simulink model "Dll_Control_AFO_V8_5_R2019b"  (R2019b)
settings: Solver=ode2  StartTime=0.0  StopTime=10  FixedStep=Ts  RelTol=1e-3
InitFcn:
  | modelDir=fileparts(get_param(bdroot,'FileName'));addpath(modelDir);rootDir=fileparts(modelDir);if isfolder(rootDir),addpath(rootDir);end;fmuDir=fullfile(rootDir,'fmu');if isfolder(fmuDir),addpath(fmuDir);end;if evalin('base','exist(''Wf0'',''var'')'),assignin('base','Wfb',evalin('base','Wf0'));end;
values from neighbouring files (symbols this model uses):
  A80 = 0.10573    [RunCtrlSysModelSHT.m]
  b11 = B(1,1)*1    [RunCtrlSysModelSHT.m]
  b21 = B(2,1)*1    [RunCtrlSysModelSHT.m]
  d31 = D(3,1)    [RunCtrlSysModelSHT.m]
  d41 = D(4,1)    [RunCtrlSysModelSHT.m]
  ExternalSecondaryAirEnabled = 0    [RunCtrlSysModelSHT.m]
  InitAir = zeros(50,1)    [RunCtrlSysModelSHT.m]
  Mkg0 = 0    [RunCtrlSysModelSHT.m]
  MkpDirectCommand = Mkp0    (= 999.278795578)    [RunCtrlSysModelSHT.m]
  MkpMax = 1200    [RunCtrlSysModelSHT.m]
  Ng0 = 38000    [RunCtrlSysModelSHT.m]
  NgMax = Ng0*1.05    (= 39900)    [RunCtrlSysModelSHT.m]
  Np0 = 20800    [RunCtrlSysModelSHT.m]
  NpDem = Np0    (= 20800)    [RunCtrlSysModelSHT.m]
  omega_u = 20    [RunCtrlSysModelSHT.m]
  power0 = 2176600    [RunCtrlSysModelSHT.m]
  RotorLoadCfg = struct(      'designNpRpm', Np0,      'designPowerW', power0,      'thetaZeroDeg', 0,      'thetaDesignDeg', 12,      'profileTorqueFraction', 0.15,      'thetaValidRangeDeg', [6, 14])    [RunCtrlSysModelSHT.m]
  RotorLoadInputMode = 'legacyPower'    [RunCtrlSysModelSHT.m]
  T45Max = 1400    [RunCtrlSysModelSHT.m]
  ThetaCommandDeg = RotorLoadCfg.thetaDesignDeg    [RunCtrlSysModelSHT.m]
  Ts = 0.025    [RunCtrlSysModelSHT.m]
  Wf0 = 0.151914044493225    (= 0.151914044493)    [RunCtrlSysModelSHT.m]
  WfMax = Wf0*2    (= 0.303828088986)    [RunCtrlSysModelSHT.m]
  WfMin = Wf0*0.01    (= 0.00151914044493)    [RunCtrlSysModelSHT.m]
  WfRateLim = 1.5    [RunCtrlSysModelSHT.m]
undefined symbols (not defined in the file or in its folder): sigbuilder_block, Wfb
libraries: simulink x10
(part 1 of 4)
settings Model: Creator=Jiangjc21  LastModifiedBy=k_liu
settings SolverCC: NumberNewtonIterations=10  SolverJacobianMethodControl=FullPerturbation
settings DataIOCC: ReturnWorkspaceOutputs=off

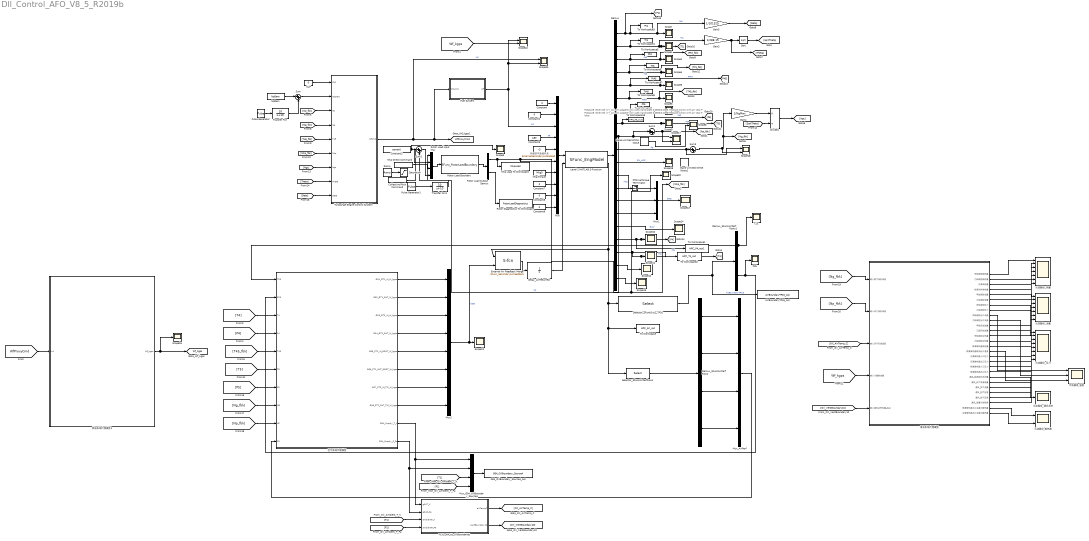
== system Dll_Control_AFO_V8_5_R2019b ==
  note: PsealA/B reserved (V7_22). Oil adapter still uses hardcoded 3.08e5/3.20e5. Replace Const with air seal P later.
  note: PsealA/B reserved (V7_22). Oil adapter still uses hardcoded 3.08e5/3.20e5. Replace Const with air seal P later.
  AirBoundaryTP16_out : ToWorkspace  VariableName=AirBoundaryTP16_out  SampleTime=-1
  Band-Limited White Noise : simulink/Sources/Band-Limited White Noise  Cov=[0.1]  Ts=Ts  seed=[23341]
  Band-Limited White Noise1 : simulink/Sources/Band-Limited White Noise  Cov=[0.1]  Ts=Ts  seed=[23341]
  CLP : Constant  Value=0
  Collective Pitch Command : Constant  Value=ThetaCommandDeg
  Constant{,1,7..9} (5 alike) : Constant  Value=0
  Constant2 : Constant  Value=power0
  Constant3 : Constant  Value=A80
  Delay_AirReturn50 : UnitDelay  InitialCondition=InitAir  SampleTime=Ts  HasFrameUpgradeWarning=on
  Demux : Demux  Outputs=20
  Demux_SFuncAirPerfRows : Demux
  Demux_SFuncAirPerfRows1 : Demux  Outputs=2
  Divide1 : Product  Inputs=*/
  External Air Feedback Merge : M-S-Function  FunctionName=SFunc_SecondaryAirFeedback
  FCN_G04_to_OilBoundaries : MATLAB Function  TreatAsAtomicUnit=on
  Fuel System : Subsystem
  G04_OilBoundary_Source4_out : ToWorkspace  VariableName=G04_OilBoundary_Source4  SampleTime=-1
  Gain3 : Gain  Gain=1/288.15
  Gain4 : Gain  Gain=1/NgMax
  Gain5 : Gain  Gain=1/101325
  Level-2 MATLAB S-Function : M-S-Function  FunctionName=SFunc_EngModel  Parameters=InitStat, InitOut, InitAir
  Mkg Torque : Constant  Value=Mkg0
  Mkp Direct Command : Constant  Value=MkpDirectCommand
  Mkp Load To Workspace : ToWorkspace  VariableName=MkpLoad  SaveFormat=Structure With Time  SampleTime=-1
  Mux : Mux  Inputs=10
  Mux1 : Mux  Inputs=3
  Mux2 : Mux  Inputs=8
  Mux_AirPerf : Mux
  Mux_G04_OilBoundary_Source4 : Mux
  NpDem : Constant  Value=NpDem
  P25 : Scope
  PTDriveTorque Terminator : Terminator
  Pulse Generator : DiscretePulseGenerator  PulseType=Time based  Amplitude=-2000  Period=100  PulseWidth=5  PhaseDelay=1
  Pulse Generator1 : DiscretePulseGenerator  PulseType=Time based  Amplitude=-4  Period=10  PulseWidth=50  PhaseDelay=1
  Ramp : simulink/Sources/Ramp  slope=-1e6  start=0  InitialOutput=0
  Rotor Diagnostics To Workspace : ToWorkspace  VariableName=RotorLoadDiagnostics  SaveFormat=Structure With Time  SampleTime=-1
  Rotor Load Boundary : M-S-Function  FunctionName=SFunc_RotorLoadBoundary  Parameters=RotorLoadInputMode,RotorLoadCfg
  Rotor Load Input Mux : Mux
  Rotor Load Output Demux : Demux  Outputs=[1 5]
  Saturation : Saturate  UpperLimit=0  LowerLimit=-power0*0.9
  Scope{,1..16,19..21} (20 alike) : Scope
  Scope{17..18,22,25} (4 alike) : Scope  NumInputPorts=2
  Selector_SFuncAirPerfRows : Selector  InputPortWidth=50  IndexOptions=Index vector (dialog)  Indices=[23 24 33 34]  OutputSizes=4
  Selector_SFuncOut2_TP16 : Selector  InputPortWidth=50  IndexOptions=Index vector (dialog)  Indices=[33 34 ]  OutputSizes=1
  Sqrt : Sqrt  SaturateOnIntegerOverflow=on
  Sum{,1..3} (4 alike) : Sum  Inputs=|++
  T25 : Scope
  To Workspace : ToWorkspace  VariableName=HPC_air_out  SaveFormat=Timeseries  SampleTime=-1
  To Workspace1 : ToWorkspace  VariableName=HPC_P4_out1  SaveFormat=Timeseries  SampleTime=-1
  To Workspace13 : ToWorkspace  VariableName=HPC_T5_out1  SaveFormat=Timeseries  SampleTime=-1
  To Workspace2 : ToWorkspace  VariableName=HPC_T4_out  SaveFormat=Timeseries  SampleTime=-1
  To Workspace3 : ToWorkspace  VariableName=Pt1  SaveFormat=Timeseries  SampleTime=-1
  To Workspace4 : ToWorkspace  VariableName=Tt1  SaveFormat=Timeseries  SampleTime=-1
  To Workspace5 : ToWorkspace  VariableName=Pt3  SaveFormat=Timeseries  SampleTime=-1
  To Workspace6 : ToWorkspace  VariableName=Tt3  SaveFormat=Timeseries  SampleTime=-1
  To Workspace7 : ToWorkspace  VariableName=Pt45  SaveFormat=Timeseries  SampleTime=-1
  To Workspace8 : ToWorkspace  VariableName=Tt45  SaveFormat=Timeseries  SampleTime=-1
  To Workspace9 : ToWorkspace  VariableName=Pt5  SaveFormat=Timeseries  SampleTime=-1
  Transfer Fcn : TransferFcn  Numerator=[10]  Denominator=[1 10]
  Transfer Fcn1 : TransferFcn  Numerator=[10]  Denominator=[1 10]
  Turboshaft Engine Control System : Subsystem
  外部空气系统开关 : Constant  Value=ExternalSecondaryAirEnabled
  滑油系统代理模型 : Subsystem
  燃油系统代理模型1 : Subsystem
  示波器组_压力 : Scope  NumInputPorts=8
  示波器组_散热器 : Scope  NumInputPorts=2
  示波器组_流量 : Scope  NumInputPorts=7
  示波器组_温度 : Scope  NumInputPorts=3
  示波器组_热量 : Scope  NumInputPorts=7
  示波器组_通风状态 : Scope
  空气系统代理模型 : Subsystem
  tag scope: WfProxyCmd=global, Wf_kgps=global
  wires:
  Demux/5 -> [P45], Scope5/1, To Workspace7/1  "Pt45"
  Mux1/1 -> Scope13/1  "beta"
  [Np_fbk] -> Turboshaft Engine Control System/3(Np)
  外部空气系统开关/1 -> Mux/5
  [Deta] -> Turboshaft Engine Control System/9(Deta)
  [Theta] -> Turboshaft Engine Control System/8(Theta)
  Gain5/1 -> [Deta]
  Demux/7 -> [P5], Scope7/1, To Workspace9/1  "Pt5"
  Divide1/1 -> [Ngc]
  [T45_fbk] -> Turboshaft Engine Control System/5(T45)
  Sqrt/1 -> [SqrtTheta]
  [Ngc] -> Turboshaft Engine Control System/7(Ngc)
  [Ng_fbk] -> Turboshaft Engine Control System/4(Ng)
  [Mkp_fbk] -> Turboshaft Engine Control System/6(Mkp)
  Demux/14 -> Mux1/2
  Demux/2 -> To Workspace4/1, [T1], Scope1/1, Gain3/1  "Tt1"
  Demux/15 -> Mux1/3
  Demux/4 -> [Tt3_fbk], Scope4/1, To Workspace6/1  "Tt3"
  Mux/1 -> Level-2 MATLAB S-Function/1
  Demux/3 -> To Workspace5/1, [Pt3_fbk], Scope2/1  "Pt3"
  Demux/6 -> Scope6/1, [T45_fbk], To Workspace8/1  "Tt45"
  Demux/1 -> [P1], Gain5/1, Scope/1, To Workspace3/1  "Pt1"
  Constant1/1 -> Mux/2
  Demux/8 -> [T5], Scope9/1, To Workspace13/1  "Tt5"
  Demux/11 -> Scope19/1  "SM_HPC"
  Constant9/1 -> Mux/10
  Constant3/1 -> Mux/4  "A8"
  Demux/10 -> Scope18/1, Sum3/1  "Ng"
  Demux/9 -> Sum2/1, Scope17/1, Rotor Load Input Mux/1  "Np"
  Gain4/1 -> Divide1/1
  Constant8/1 -> Mux/9
  Gain3/1 -> [Theta], Sqrt/1
  [SqrtTheta] -> Divide1/2
  Demux/13 -> Mux1/1
  Constant/1 -> Mux/1
  CLP/1 -> Turboshaft Engine Control System/1(CLP)
  Constant7/1 -> Mux/8
  Band-Limited White Noise/1 -> Scope8/1
  Sum2/1 -> Scope17/2, [Np_fbk]
  Sum3/1 -> Scope18/2, Gain4/1, [Ng_fbk]
  Sum/1 -> Turboshaft Engine Control System/2(NpDem)
  Fuel System/1(Wf) -> Mux/3, Scope22/1, Scope25/2  "Wf"
  NpDem/1 -> Sum/1
  Pulse Generator/1 -> Transfer Fcn/1
  Pulse Generator1/1 -> Transfer Fcn1/1
  Ramp/1 -> Saturation/1
  Transfer Fcn/1 -> Sum/2
  Demux/16 -> Scope14/1  "Error"
  Demux/17 -> [P4], Scope10/1, To Workspace1/1  "Pt4"
  Demux/18 -> [T4], Scope11/1, To Workspace2/1  "Tt4"
  Demux/19 -> Scope12/1
  Demux/20 -> Scope15/1
  燃油系统代理模型1/1(Wf_kgps) -> [Wf_kgps], Scope16/1
  Level-2 MATLAB S-Function/1 -> Demux/1
  Level-2 MATLAB S-Function/2 -> Selector_SFuncOut2_TP16/1, To Workspace/1, Selector_SFuncAirPerfRows/1, External Air Feedback Merge/1
  Selector_SFuncOut2_TP16/1 -> AirBoundaryTP16_out/1, Demux_SFuncAirPerfRows1/1  "AirBoundaryTP16"
  Demux_SFuncAirPerfRows1/2 -> 空气系统代理模型/2(P25), P25/1
  [T4] -> 空气系统代理模型/3(T4)
  [P4] -> 空气系统代理模型/4(P4)
  [T45_fbk] -> 空气系统代理模型/5(T45)
  [T5] -> 空气系统代理模型/6(T5)
  [P5] -> 空气系统代理模型/7(P5)
  [Ng_fbk] -> 空气系统代理模型/8(NG)
  [Np_fbk] -> 空气系统代理模型/9(NP)
  空气系统代理模型/1(G01_GT1_IN_W_kgps) -> Mux2/1
  空气系统代理模型/2(G02_GT1_OUT_W_kgps) -> Mux2/2
  空气系统代理模型/3(G03_GT2_IN_W_kgps) -> Mux2/3
  空气系统代理模型/4(G04_GT2_OUT_W_kgps) -> Mux2/4
  空气系统代理模型/5(G05_PT1_IN_ROOT_W_kgps) -> Mux2/5
  空气系统代理模型/6(G06_PT1_OUT_ROOT_W_kgps) -> Mux2/6
  空气系统代理模型/7(G07_PT2_IN_TIP_W_kgps) -> Mux2/7
  空气系统代理模型/8(G08_PT2_OUT_TIP_W_kgps) -> Mux2/8
  Mux2/1 -> Scope21/1, External Air Feedback Merge/2  "beta"
  Selector_SFuncAirPerfRows/1 -> Demux_SFuncAirPerfRows/1
  Demux_SFuncAirPerfRows/2 -> Mux_AirPerf/2
  Delay_AirReturn50/1 -> Level-2 MATLAB S-Function/2
  Demux_SFuncAirPerfRows/1 -> Mux_AirPerf/1
  Demux_SFuncAirPerfRows/3 -> Mux_AirPerf/3
  Demux_SFuncAirPerfRows/4 -> Mux_AirPerf/4
  Mux_AirPerf/1 -> 空气系统代理模型/10(25)
  [Ng_fbk] -> 滑油系统代理模型/1(输入燃气涡轮转速)
  [Np_fbk] -> 滑油系统代理模型/2(输入动力涡轮转速)
  [Wf_kgps] -> 滑油系统代理模型/4(输入计量燃油量)
  [T1] -> FCN_G04_to_OilBoundaries/3(ambientT_K)
  [P1] -> FCN_G04_to_OilBoundaries/4(ambientP_Pa)
  FCN_G04_to_OilBoundaries/1(airTempC) -> [Oil_AirTemp_C]
  FCN_G04_to_OilBoundaries/2(ventBoundary10) -> [Oil_VentBoundary10]
  [T1] -> Mux_G04_OilBoundary_Source4/3
  [P1] -> Mux_G04_OilBoundary_Source4/4
  Mux_G04_OilBoundary_Source4/1 -> G04_OilBoundary_Source4_out/1
  [Oil_AirTemp_C] -> 滑油系统代理模型/3(输入空气系统温度)
  [Oil_VentBoundary10] -> 滑油系统代理模型/5(输入通风边界向量_PaK)
  空气系统代理模型/10(G04_Supply_P_Pa) -> Mux_G04_OilBoundary_Source4/2, FCN_G04_to_OilBoundaries/2(g04P_Pa)
  空气系统代理模型/9(G04_Supply_T_K) -> FCN_G04_to_OilBoundaries/1(g04T_K), Mux_G04_OilBoundary_Source4/1
  滑油系统代理模型/1(甲轴承腔换热量) -> 示波器组_热量/1
  滑油系统代理模型/2(乙轴承腔换热量) -> 示波器组_热量/2
  滑油系统代理模型/3(空滑换热量) -> 示波器组_热量/3
  滑油系统代理模型/4(机匣附件换热量) -> 示波器组_热量/4
  滑油系统代理模型/13(甲轴承腔生热量) -> 示波器组_热量/5
  滑油系统代理模型/14(乙轴承腔生热量) -> 示波器组_热量/6
  滑油系统代理模型/15(燃滑散热器换热量) -> 示波器组_热量/7
  滑油系统代理模型/5(甲轴承腔流量) -> 示波器组_流量/1
  滑油系统代理模型/6(乙轴承腔流量) -> 示波器组_流量/2
  滑油系统代理模型/11(甲腔回油流量) -> 示波器组_流量/3
  滑油系统代理模型/12(乙腔回油流量) -> 示波器组_流量/4
  滑油系统代理模型/22(通风_封严泄漏流量) -> 示波器组_流量/5
  滑油系统代理模型/23(通风_排气流量) -> 示波器组_流量/6
  滑油系统代理模型/26(通风_质量守恒残差) -> 示波器组_流量/7
  滑油系统代理模型/7(甲轴承腔压力) -> 示波器组_压力/1
  滑油系统代理模型/8(乙轴承腔压力) -> 示波器组_压力/2
  滑油系统代理模型/17(空滑散热器入口压力) -> 示波器组_压力/3
  滑油系统代理模型/18(空滑散热器出口压力) -> 示波器组_压力/4
  滑油系统代理模型/19(燃滑散热器入口压力) -> 示波器组_压力/5
  滑油系统代理模型/20(燃滑散热器出口压力) -> 示波器组_压力/6
  滑油系统代理模型/24(通风_封严压差) -> 示波器组_压力/7
  滑油系统代理模型/25(通风_排气压差) -> 示波器组_压力/8
  滑油系统代理模型/9(甲轴承腔出口油温) -> 示波器组_温度/1
  滑油系统代理模型/10(乙轴承腔出口油温) -> 示波器组_温度/2
  滑油系统代理模型/16(燃滑散热器燃油出口温度) -> 示波器组_温度/3
  滑油系统代理模型/21(通风_轴承腔状态向量) -> 示波器组_通风状态/1
  滑油系统代理模型/27(燃滑散热器出口油温与散热量) -> 示波器组_散热器/1
  滑油系统代理模型/28(空滑散热器出口油温与散热量) -> 示波器组_散热器/2
  Constant2/1 -> Rotor Load Input Mux/2, Scope3/1
  Mkp Direct Command/1 -> Rotor Load Input Mux/3
  Collective Pitch Command/1 -> Sum1/1
  Transfer Fcn1/1 -> Sum1/2
  Sum1/1 -> Rotor Load Input Mux/4
  Rotor Load Input Mux/1 -> Rotor Load Boundary/1
  Rotor Load Boundary/1 -> Rotor Load Output Demux/1
  Rotor Load Output Demux/1 -> [Mkp_fbk], Scope20/1, Mux/6, Mkp Load To Workspace/1
  Rotor Load Output Demux/2 -> Rotor Diagnostics To Workspace/1
  Demux/12 -> PTDriveTorque Terminator/1  "Mkp"
  Mkg Torque/1 -> Mux/7
  External Air Feedback Merge/1 -> Delay_AirReturn50/1
  Turboshaft Engine Control System/1(Wfcmd) -> [WfProxyCmd], Fuel System/1(Wf_cmd), Scope25/1  "Wf"
  Demux_SFuncAirPerfRows1/1 -> T25/1, 空气系统代理模型/1(T25)
  [WfProxyCmd] -> 燃油系统代理模型1/1(In1)
  [Wf_kgps] -> Scope22/2

== system Dll_Control_AFO_V8_5_R2019b/Fuel System ==
  Wf_cmd : Inport
  Constant : Constant  Value=Wf0
  Gain3 : Gain  Gain=25
  Integrator3 : Integrator  InitialConditionSource=external  InitialCondition=Wfb  LimitOutput=on  UpperSaturationLimit=WfMax  LowerSaturationLimit=WfMin
  Saturation : Saturate  UpperLimit=WfRateLim  LowerLimit=-WfRateLim
  Sum3 : Sum  Inputs=|+-
  Wf : Outport
  wires:
  Saturation/1 -> Integrator3/1
  Gain3/1 -> Saturation/1
  Sum3/1 -> Gain3/1
  Wf_cmd/1 -> Sum3/1
  Integrator3/1 -> Wf/1, Sum3/2
  Constant/1 -> Integrator3/2

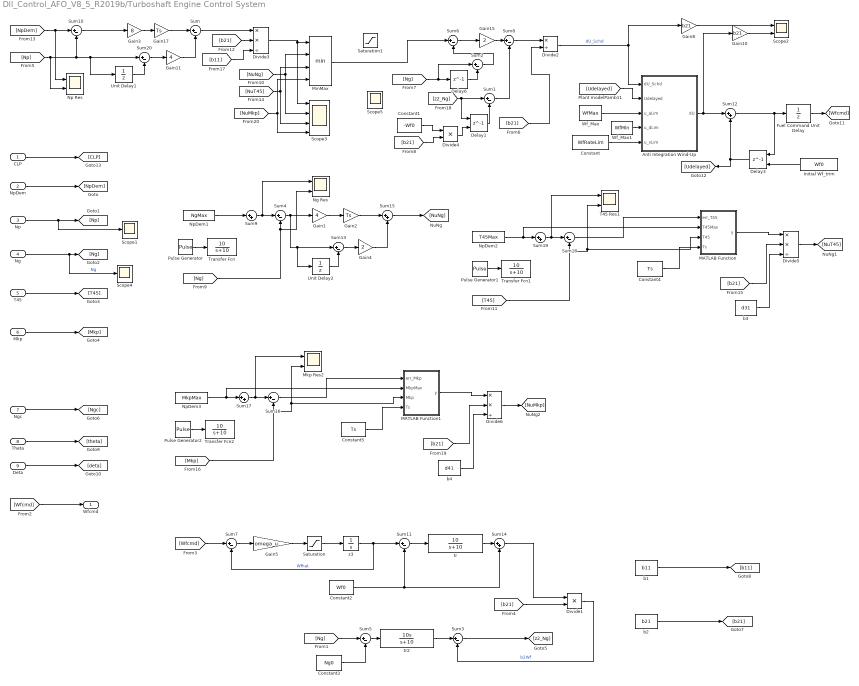
== system Dll_Control_AFO_V8_5_R2019b/Turboshaft Engine Control System ==
  CLP : Inport
  NpDem : Inport  Port=2
  Np : Inport  Port=3
  Ng : Inport  Port=4
  T45 : Inport  Port=5
  Mkp : Inport  Port=6
  Ngc : Inport  Port=7
  Theta : Inport  Port=8
  Deta : Inport  Port=9
  Anti Integration Wind-Up : MATLAB Function  TreatAsAtomicUnit=on
  Constant : Constant  Value=WfRateLim
  Constant1 : Constant  Value=-Wf0
  Constant2 : Constant  Value=Wf0
  Constant3 : Constant  Value=Ng0
  Constant4 : Constant  Value=Ts
  Constant5 : Constant  Value=Ts
  Delay1 : Delay  DelayLength=1  InitialConditionSource=Input port  InitialCondition=Ng0  SampleTime=Ts
      settings: InputPortMap=u0,p4
  Delay3 : Delay  DelayLength=1  InitialConditionSource=Input port  InitialCondition=Wfb  SampleTime=Ts
      settings: InputPortMap=u0,p4
  Delay6 : Delay  DelayLength=1  InitialCondition=Ng0  SampleTime=Ts
  Divide1 : Product  Inputs=**
  Divide2 : Product  Inputs=*/
  Divide3 : Product  Inputs=**/
  Divide4 : Product  Inputs=**
  Divide5 : Product  Inputs=**/
  Divide6 : Product  Inputs=**/
  Fuel Command Unit Delay : UnitDelay  InitialCondition=Wf0  SampleTime=Ts  HasFrameUpgradeWarning=on
  Gain1 : Gain  Gain=4
  Gain10 : Gain  Gain=b21
  Gain11 : Gain  Gain=4
  Gain15 : Gain  Gain=2
  Gain17 : Gain  Gain=Ts
  Gain2 : Gain  Gain=Ts
  Gain3 : Gain  Gain=8
  Gain4 : Gain  Gain=2
  Gain5 : Gain  Gain=omega_u
  Gain8 : Gain  Gain=b21
  Initial Wf_trim : Constant  Value=Wf0
  MATLAB Function : MATLAB Function  TreatAsAtomicUnit=on
  MATLAB Function1 : MATLAB Function  TreatAsAtomicUnit=on
  MinMax : MinMax  Inputs=4
  Mkp Res2 : Scope  NumInputPorts=2
  Ng Res : Scope  NumInputPorts=2
  Np Res : Scope  NumInputPorts=2
  NpDem1 : Constant  Value=NgMax
  NpDem2 : Constant  Value=T45Max
  NpDem3 : Constant  Value=MkpMax
  Pulse Generator : DiscretePulseGenerator  PulseType=Time based  Amplitude=-200  Period=10  PulseWidth=40  PhaseDelay=2
  Pulse Generator1 : DiscretePulseGenerator  PulseType=Time based  Amplitude=-5  Period=10  PulseWidth=40  PhaseDelay=2
  Pulse Generator2 : DiscretePulseGenerator  PulseType=Time based  Amplitude=-50  Period=10  PulseWidth=40  PhaseDelay=2
  Saturation : Saturate  UpperLimit=WfRateLim  LowerLimit=-WfRateLim
  Saturation1 : Saturate  UpperLimit=1000  LowerLimit=-1000
  Scope1 : Scope
  Scope2 : Scope  NumInputPorts=2
  Scope3 : Scope  NumInputPorts=4
  Scope4 : Scope
  Scope5 : Scope  NumInputPorts=2
  Sum{,1..8,10..11,13,16,18,20} (15 alike) : Sum  Inputs=|+-
  Sum{9,12,14..15,17,19} (6 alike) : Sum  Inputs=|++
  T45 Res1 : Scope  NumInputPorts=2
  Transfer Fcn : TransferFcn  Numerator=[10]  Denominator=[1 10]
  Transfer Fcn1 : TransferFcn  Numerator=[10]  Denominator=[1 10]
  Transfer Fcn2 : TransferFcn  Numerator=[10]  Denominator=[1 10]
  Unit Delay1 : UnitDelay  InitialCondition=Np0  SampleTime=-1  HasFrameUpgradeWarning=on
  Unit Delay2 : UnitDelay  InitialCondition=NgMax-Ng0  SampleTime=-1  HasFrameUpgradeWarning=on
  Wf_Max : Constant  Value=WfMax
  Wf_Max1 : Constant  Value=WfMin
  b1 : Constant  Value=b11
  b2 : Constant  Value=b21
  b3 : Constant  Value=d31
  b4 : Constant  Value=d41
  tr : TransferFcn  Numerator=[10]  Denominator=[1 10]
  tr2 : TransferFcn  Numerator=[10 0]  Denominator=[1 10]
  z3 : Integrator  InitialCondition=Wf0
  Wfcmd : Outport
  wires:
  NpDem/1 -> [NpDem]
  Np/1 -> Scope1/1, [Np]
  Ng/1 -> Scope4/1, [Ng]  "Ng"
  T45/1 -> [T45]
  Mkp/1 -> [Mkp]
  [Wfcmd] -> Wfcmd/1
  Ngc/1 -> [Ngc]
  Theta/1 -> [theta]
  Deta/1 -> [deta]
  Delay3/1 -> [Udelayed], Sum12/2
  Initial Wf_trim/1 -> Delay3/2
  Wf_Max1/1 -> Anti Integration Wind-Up/4(u_dLim)
  Wf_Max/1 -> Anti Integration Wind-Up/3(u_aLim)
  CLP/1 -> [CLP]
  z3/1 -> Sum11/1, Sum7/2  "Wfhat"
  Sum7/1 -> Gain5/1
  Constant/1 -> Anti Integration Wind-Up/5(u_vLim)
  [b21] -> Divide2/2
  Anti Integration Wind-Up/1(dU) -> Gain10/1, Sum12/1
  Constant2/1 -> Sum14/2, Sum11/2
  Sum11/1 -> tr/1
  tr/1 -> Sum14/1
  [NpDem] -> Sum10/1, Np Res/1
  Sum8/1 -> Divide2/1
  Gain5/1 -> Saturation/1
  Saturation/1 -> z3/1
  [Wfcmd] -> Sum7/1
  [Udelayed] -> Anti Integration Wind-Up/2(Udelayed)
  Gain8/1 -> Scope2/1
  Gain10/1 -> Scope2/2
  [Np] -> Sum20/1, Unit Delay1/1, Sum10/2, Np Res/2
  tr2/1 -> Sum3/1
  [b21] -> Divide1/2
  Constant3/1 -> Sum5/2
  [Ng] -> Sum5/1
  Sum5/1 -> tr2/1
  Divide1/1 -> Sum3/2  "b2Wf"
  Sum3/1 -> [z2_Ng]
  Sum14/1 -> Divide1/1
  Sum/1 -> Divide3/1
  Gain3/1 -> Gain17/1
  Sum6/1 -> Gain15/1
  Sum20/1 -> Gain11/1
  Unit Delay1/1 -> Sum20/2
  [b21] -> Divide3/2
  [b11] -> Divide3/3
  Divide2/1 -> Anti Integration Wind-Up/1(dU_Schd), Gain8/1  "dU_Schd"
  Gain15/1 -> Sum8/1
  Gain17/1 -> Sum/1
  Gain11/1 -> Sum/2
  [Ng] -> Sum2/1, Delay6/1
  Delay6/1 -> Sum2/2
  b1/1 -> [b11]
  b2/1 -> [b21]
  [z2_Ng] -> Sum1/1, Delay1/1
  Delay1/1 -> Sum1/2
  Constant1/1 -> Divide4/1
  [b21] -> Divide4/2
  Divide4/1 -> Delay1/2
  Sum12/1 -> Fuel Command Unit Delay/1, Delay3/1
  Fuel Command Unit Delay/1 -> [Wfcmd]
  Pulse Generator/1 -> Transfer Fcn/1
  NpDem1/1 -> Sum9/1
  Sum9/1 -> Sum4/1, Ng Res/1
  Gain1/1 -> Gain2/1
  Unit Delay2/1 -> Sum13/2
  Sum13/1 -> Gain4/1
  Sum4/1 -> Unit Delay2/1, Sum13/1, Gain1/1
  Gain2/1 -> Sum15/1
  Divide3/1 -> Scope3/1, MinMax/1
  [NuNg] -> MinMax/2, Scope3/2
  Pulse Generator1/1 -> Transfer Fcn1/1
  NpDem2/1 -> MATLAB Function/2(T45Max), Sum19/1
  Sum19/1 -> Sum18/1, T45 Res1/1
  [T45] -> MATLAB Function/3(T45), T45 Res1/2, Sum18/2
  [b21] -> Divide5/2
  b3/1 -> Divide5/3
  Sum2/1 -> Sum6/2
  Sum1/1 -> Sum8/2
  [NuT45] -> Scope3/3, MinMax/3
  [Ng] -> Ng Res/2, Sum4/2
  Gain4/1 -> Sum15/2
  Sum18/1 -> MATLAB Function/1(err_T45)
  Divide5/1 -> [NuT45]
  MATLAB Function/1(y) -> Divide5/1
  Constant4/1 -> MATLAB Function/4(Ts)
  Sum15/1 -> [NuNg]
  Pulse Generator2/1 -> Transfer Fcn2/1
  Constant5/1 -> MATLAB Function1/4(Ts)
  MATLAB Function1/1(y) -> Divide6/1
  b4/1 -> Divide6/3
  Sum17/1 -> Sum16/1, Mkp Res2/1
  Sum16/1 -> MATLAB Function1/1(err_Mkp)
  NpDem3/1 -> MATLAB Function1/2(MkpMax), Sum17/1
  Divide6/1 -> [NuMkp]
  [b21] -> Divide6/2
  [Mkp] -> MATLAB Function1/3(Mkp), Mkp Res2/2, Sum16/2
  [NuMkp] -> MinMax/4, Scope3/4
  MinMax/1 -> Sum6/1
  Sum10/1 -> Gain3/1

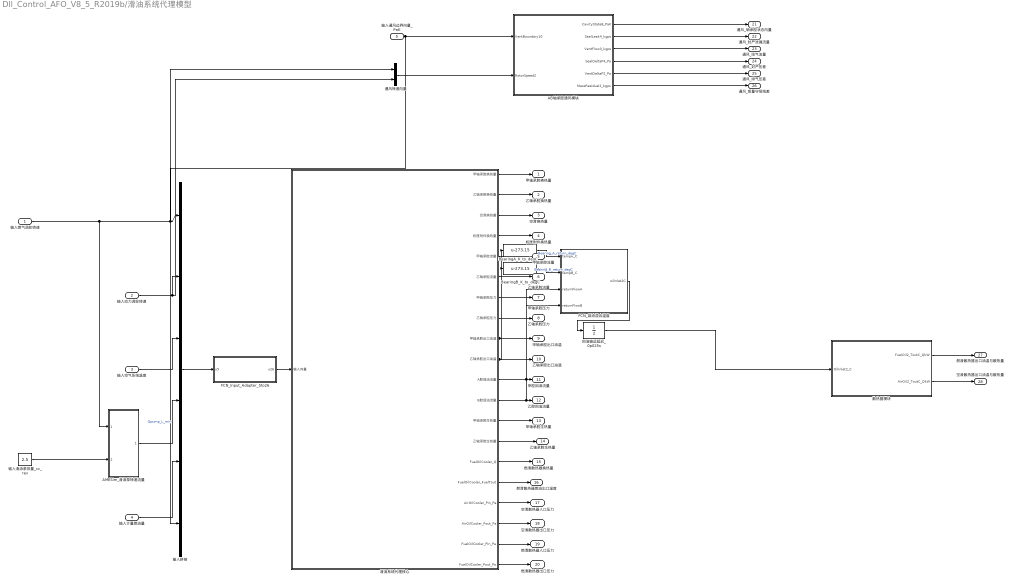
== system Dll_Control_AFO_V8_5_R2019b/滑油系统代理模型 ==
  输入燃气涡轮转速 : Inport
  输入动力涡轮转速 : Inport  Port=2
  输入空气系统温度 : Inport  Port=3
  输入计量燃油量 : Inport  Port=4
  输入通风边界向量_PaK : Inport  Port=5  PortDimensions=10
  AB轴承腔通风模块 : Subsystem
  AMESim_滑油泵转速流量 : Subsystem
  BearingA_K_to_degC : Bias  Description=轴承出口绝对温度K仅在进入摄氏度混温接口前换算，不改变原始输出单位。  Bias=-273.15
  BearingB_K_to_degC : Bias  Description=轴承出口绝对温度K仅在进入摄氏度混温接口前换算，不改变原始输出单位。  Bias=-273.15
  FCN_Input_Adapter_5to26 : MATLAB Function  TreatAsAtomicUnit=on
  FCN_回油混合温度 : MATLAB Function  TreatAsAtomicUnit=on
  回油输运延迟_0p025s : UnitDelay  InitialCondition=[130;130]  SampleTime=0.025  HasFrameUpgradeWarning=on
  散热器模块 : Subsystem
  滑油系统代理核心 : Subsystem
  输入拼接 : Mux  Inputs=6
  输入滑油泵排量_cc_rev : Constant  Value=2.5
  通风转速向量 : Mux  Inputs=2
  甲轴承腔换热量 : Outport
  乙轴承腔换热量 : Outport  Port=2
  空滑换热量 : Outport  Port=3
  机匣附件换热量 : Outport  Port=4
  甲轴承腔流量 : Outport  Port=5
  乙轴承腔流量 : Outport  Port=6
  甲轴承腔压力 : Outport  Port=7
  乙轴承腔压力 : Outport  Port=8
  甲轴承腔出口油温 : Outport  Port=9
  乙轴承腔出口油温 : Outport  Port=10
  甲腔回油流量 : Outport  Port=11
  乙腔回油流量 : Outport  Port=12
  甲轴承腔生热量 : Outport  Port=13
  乙轴承腔生热量 : Outport  Port=14
  燃滑散热器换热量 : Outport  Port=15
  燃滑散热器燃油出口温度 : Outport  Port=16
  空滑散热器入口压力 : Outport  Port=17
  空滑散热器出口压力 : Outport  Port=18
  燃滑散热器入口压力 : Outport  Port=19
  燃滑散热器出口压力 : Outport  Port=20
  通风_轴承腔状态向量 : Outport  Port=21  PortDimensions=8
  通风_封严泄漏流量 : Outport  Port=22  PortDimensions=4
  通风_排气流量 : Outport  Port=23  PortDimensions=3
  通风_封严压差 : Outport  Port=24  PortDimensions=4
  通风_排气压差 : Outport  Port=25  PortDimensions=2
  通风_质量守恒残差 : Outport  Port=26  PortDimensions=2
  燃滑散热器出口油温与散热量 : Outport  Port=27  PortDimensions=2
  空滑散热器出口油温与散热量 : Outport  Port=28  PortDimensions=2
  wires:
  滑油系统代理核心/18(AirOilCooler_Pout_Pa) -> 空滑散热器出口压力/1
  输入拼接/1 -> FCN_Input_Adapter_5to26/1(u5)
  AB轴承腔通风模块/6(MassResidual2_kgps) -> 通风_质量守恒残差/1
  滑油系统代理核心/1(甲轴承腔换热量) -> 甲轴承腔换热量/1
  滑油系统代理核心/14(乙轴承腔生热量) -> 乙轴承腔生热量/1
  滑油系统代理核心/17(AirOilCooler_Pin_Pa) -> 空滑散热器入口压力/1
  滑油系统代理核心/2(乙轴承腔换热量) -> 乙轴承腔换热量/1
  输入计量燃油量/1 -> 输入拼接/5
  通风转速向量/1 -> AB轴承腔通风模块/2(RotorSpeed2)
  AB轴承腔通风模块/5(VentDeltaP2_Pa) -> 通风_排气压差/1
  滑油系统代理核心/6(乙轴承腔流量) -> 乙轴承腔流量/1
  滑油系统代理核心/10(乙轴承腔出口油温) -> 乙轴承腔出口油温/1, BearingB_K_to_degC/1
  滑油系统代理核心/12(B腔回油流量) -> 乙腔回油流量/1, FCN_回油混合温度/4(returnFlowB)
  输入动力涡轮转速/1 -> 输入拼接/2, 通风转速向量/2
  滑油系统代理核心/11(A腔回油流量) -> 甲腔回油流量/1, FCN_回油混合温度/3(returnFlowA)
  FCN_Input_Adapter_5to26/1(u26) -> 滑油系统代理核心/1(输入向量)
  滑油系统代理核心/15(FuelOilCooler_Q) -> 燃滑散热器换热量/1
  滑油系统代理核心/8(乙轴承腔压力) -> 乙轴承腔压力/1
  滑油系统代理核心/4(机匣附件换热量) -> 机匣附件换热量/1
  输入燃气涡轮转速/1 -> 通风转速向量/1, 输入拼接/1, AMESim_滑油泵转速流量/1(Ng_rpm)
  滑油系统代理核心/19(FuelOilCooler_Pin_Pa) -> 燃滑散热器入口压力/1
  输入滑油泵排量_cc_rev/1 -> AMESim_滑油泵转速流量/2(泵排量_cc_rev)
  输入空气系统温度/1 -> 输入拼接/3
  滑油系统代理核心/16(FuelOilCooler_FuelTout) -> 燃滑散热器燃油出口温度/1
  输入通风边界向量_PaK/1 -> AB轴承腔通风模块/1(VentBoundary10), 输入拼接/6
  AMESim_滑油泵转速流量/1(Qpump_L_min) -> 输入拼接/4  "Qpump_L_min"
  散热器模块/2(AirOil2_ToutC_QkW) -> 空滑散热器出口油温与散热量/1
  滑油系统代理核心/7(甲轴承腔压力) -> 甲轴承腔压力/1
  滑油系统代理核心/9(甲轴承腔出口油温) -> 甲轴承腔出口油温/1, BearingA_K_to_degC/1
  滑油系统代理核心/3(空滑换热量) -> 空滑换热量/1
  AB轴承腔通风模块/3(VentFlow3_kgps) -> 通风_排气流量/1
  滑油系统代理核心/13(甲轴承腔生热量) -> 甲轴承腔生热量/1
  AB轴承腔通风模块/2(SealLeak4_kgps) -> 通风_封严泄漏流量/1
  滑油系统代理核心/5(甲轴承腔流量) -> 甲轴承腔流量/1
  AB轴承腔通风模块/1(CavityState8_PaK) -> 通风_轴承腔状态向量/1
  散热器模块/1(FuelOil2_ToutC_QkW) -> 燃滑散热器出口油温与散热量/1
  AB轴承腔通风模块/4(SealDeltaP4_Pa) -> 通风_封严压差/1
  滑油系统代理核心/20(FuelOilCooler_Pout_Pa) -> 燃滑散热器出口压力/1
  FCN_回油混合温度/1(oilInlet2C) -> 回油输运延迟_0p025s/1
  回油输运延迟_0p025s/1 -> 散热器模块/1(OilInlet2_C)
  BearingA_K_to_degC/1 -> FCN_回油混合温度/1(tempA_C)  "Bearing_A_return_degC"
  BearingB_K_to_degC/1 -> FCN_回油混合温度/2(tempB_C)  "Bearing_B_return_degC"

== system Dll_Control_AFO_V8_5_R2019b/燃油系统代理模型1 ==
  note: 油压Mpa
  note: 停车信号0/1
  note: 计量位移输出m
  note: 闭锁信号0/1
  note: 导叶输入
  note: 计量输入
  note: 压差输入
  note: 停车输入
  note: 导叶位移输出m
  note: 位移信号/m
  note: 位移信号/m
  note: 计量流量输出kg/s
  note: 闭锁信号0/1
  In1 : Inport
  Constant5 : Constant  Value=0.38
  FuelProxy_Lmin_to_kgps : Gain
  Mux3 : Mux  Inputs=2
  Mux4 : Mux  Inputs=2
  Scope{1..4,12} (5 alike) : Scope
  Signal Builder : Subsystem  Tag=STV Subsys  LoadFcn=sigbuilder_block('load');  StartFcn=sigbuilder_block('start');  StopFcn=sigbuilder_block('stop');  ClipboardFcn=sigbuilder_block('clipboard');  mask(Sigbuilder block){tuvar=[0:10]}
      mask help: Simulink:masks:SigbuilderBlock_MD
      mask init:
      | if ~strcmp(get_param(bdroot(gcbh),'SimulationStatus'),'stopped') tuvar = sigbuilder_block('maskInit'); end
      settings: CopyFcn=sigbuilder_block('copy');  DeleteFcn=sigbuilder_block('delete');  ModelCloseFcn=sigbuilder_block('modelClose');  PreSaveFcn=sigbuilder_block('preSave');  PauseFcn=sigbuilder_block('pause');  ContinueFcn=sigbuilder_block('continue');  NameChangeFcn=sigbuilder_block('namechange');  OpenFcn=sigbuilder_block('open',[1280 36 1280 630 ]);  CloseFcn=sigbuilder_block('close');
      mask Display: plot(0, 0, 100, 100,[2, 2, 32, 32, 2], [68, 8, 8, 68, 68],[32, 2], [38, 38], [32, 19, 2],[53, 60, 44], [32, 17, 17, 2],[16, 16, 31, 31]);txt = getActiveGroup(gcbh);text(2, 100, txt,'verticalAlignment', 'top');
  Signal Builder1 : Subsystem  Tag=STV Subsys  LoadFcn=sigbuilder_block('load');  StartFcn=sigbuilder_block('start');  StopFcn=sigbuilder_block('stop');  ClipboardFcn=sigbuilder_block('clipboard');  mask(Sigbuilder block){tuvar=[0:10]}
      mask help: Simulink:masks:SigbuilderBlock_MD
      mask init:
      | if ~strcmp(get_param(bdroot(gcbh),'SimulationStatus'),'stopped') tuvar = sigbuilder_block('maskInit'); end
      settings: CopyFcn=sigbuilder_block('copy');  DeleteFcn=sigbuilder_block('delete');  ModelCloseFcn=sigbuilder_block('modelClose');  PreSaveFcn=sigbuilder_block('preSave');  PauseFcn=sigbuilder_block('pause');  ContinueFcn=sigbuilder_block('continue');  NameChangeFcn=sigbuilder_block('namechange');  OpenFcn=sigbuilder_block('open',[1309.5 228 550.5 363 ]);  CloseFcn=sigbuilder_block('close');
      mask Display: plot(0, 0, 100, 100,[2, 2, 32, 32, 2], [68, 8, 8, 68, 68],[32, 2], [38, 38], [32, 19, 2],[53, 60, 44], [32, 17, 17, 2],[16, 16, 31, 31]);txt = getActiveGroup(gcbh);text(2, 100, txt,'verticalAlignment', 'top');
  Step : Step  Time=15  After=0  SampleTime=0
  Step1 : Step  Time=6  SampleTime=0
  Step2 : Step  Time=10  After=0  SampleTime=0
  Terminator : Terminator
  Terminator1 : Terminator
  Terminator2 : Terminator
  Wf_to_xm_inverse : Subsystem
  燃油系统代理模型 : Subsystem
  Wf_kgps : Outport
  wires:
  燃油系统代理模型/1(xm) -> Mux3/2, Terminator1/1
  Signal Builder/1(Signal 1) -> Mux3/1, 燃油系统代理模型/3(In3)
  Step/1 -> 燃油系统代理模型/2(In2)
  Mux3/1 -> Scope2/1, FuelProxy_Lmin_to_kgps/1
  Constant5/1 -> 燃油系统代理模型/1(In1)
  Step2/1 -> 燃油系统代理模型/7(In6)
  Signal Builder1/1(Signal 1) -> Mux4/1, 燃油系统代理模型/6(In5)
  Step1/1 -> 燃油系统代理模型/5(In4)
  燃油系统代理模型/3(xd) -> Mux4/2, Terminator2/1
  Mux4/1 -> Scope12/1
  In1/1 -> Wf_to_xm_inverse/1(Wf_cmd_kgps)
  Wf_to_xm_inverse/1(xm_cmd_m) -> Scope3/1, 燃油系统代理模型/4(In7)
  FuelProxy_Lmin_to_kgps/1 -> Scope1/1
  燃油系统代理模型/2(Wf) -> Terminator/1, Scope4/1, Wf_kgps/1

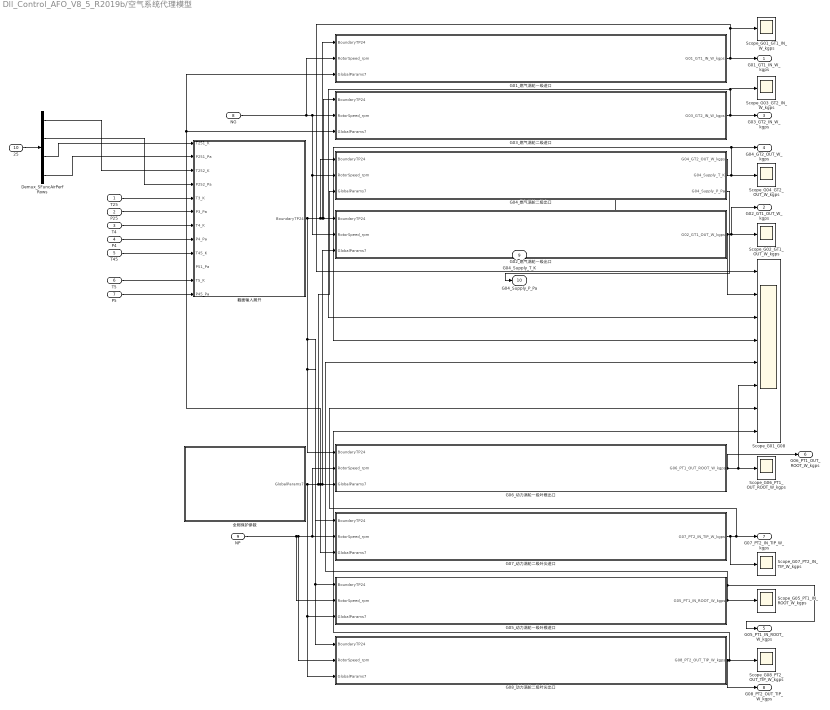
== system Dll_Control_AFO_V8_5_R2019b/空气系统代理模型 ==
  T25 : Inport
  P25 : Inport  Port=2
  T4 : Inport  Port=3
  P4 : Inport  Port=4
  T45 : Inport  Port=5
  T5 : Inport  Port=6
  P5 : Inport  Port=7
  NG : Inport  Port=8
  NP : Inport  Port=9
  25 : Inport  Port=10
  Demux_SFuncAirPerfRows : Demux
  G01_燃气涡轮一级进口 : Subsystem  Description=|
      | G01_燃气涡轮一级进口
      | Centrifugal supply through preswirl/restrictor and GT1 vane cooling.
  G02_燃气涡轮一级出口 : Subsystem  Description=|
      | G02_燃气涡轮一级出口
      | GT1 rear cavity, casing branch and seal return to GT1 outlet.
  G03_燃气涡轮二级进口 : Subsystem  Description=|
      | G03_燃气涡轮二级进口
      | GT2 front cavity and vane feed before the GT2 inlet section.
  G04_燃气涡轮二级出口 : Subsystem  Description=|
      | G04_燃气涡轮二级出口
      | GT2 casing serial restriction and outlet return.
  G05_动力涡轮一级叶根进口 : Subsystem  Description=|
      | G05_动力涡轮一级叶根进口
      | Axial-root supply, distribution hole and PT1 cavity/vane branch.
  G06_动力涡轮一级叶根出口 : Subsystem  Description=|
      | G06_动力涡轮一级叶根出口
      | Special capillar_14 - thermal cavity - orifice_45 PT1 outlet path.
  G07_动力涡轮二级叶尖进口 : Subsystem  Description=|
      | G07_动力涡轮二级叶尖进口
      | Axial-tip supply through four-port cavity and seal to PT2 inlet.
  G08_动力涡轮二级叶尖出口 : Subsystem  Description=|
      | G08_动力涡轮二级叶尖出口
      | Tip cavity through serial outlet restrictions/seal to PT2 outlet.
  Scope_G01_G08 : Scope  NumInputPorts=8
  Scope_G01_GT1_IN_W_kgps : Scope
  Scope_G02_GT1_OUT_W_kgps : Scope
  Scope_G03_GT2_IN_W_kgps : Scope
  Scope_G04_GT2_OUT_W_kgps : Scope
  Scope_G05_PT1_IN_ROOT_W_kgps : Scope
  Scope_G06_PT1_OUT_ROOT_W_kgps : Scope
  Scope_G07_PT2_IN_TIP_W_kgps : Scope
  Scope_G08_PT2_OUT_TIP_W_kgps : Scope
  全局保护参数 : Subsystem  Description=双击常量块调整全局气体性质与保护限幅。
  截面输入展开 : Subsystem  Description=将唯一截面 T1/P1..T5/P5 展开为原 12 边界 Amesim 顺序。同名截面共用输入；pn_source_17/18 由截面算术平均得到。
  G01_GT1_IN_W_kgps : Outport
  G02_GT1_OUT_W_kgps : Outport  Port=2
  G03_GT2_IN_W_kgps : Outport  Port=3
  G04_GT2_OUT_W_kgps : Outport  Port=4
  G05_PT1_IN_ROOT_W_kgps : Outport  Port=5
  G06_PT1_OUT_ROOT_W_kgps : Outport  Port=6
  G07_PT2_IN_TIP_W_kgps : Outport  Port=7
  G08_PT2_OUT_TIP_W_kgps : Outport  Port=8
  G04_Supply_T_K : Outport  Port=9
  G04_Supply_P_Pa : Outport  Port=10
  wires:
  G02_燃气涡轮一级出口/1(G02_GT1_OUT_W_kgps) -> Scope_G02_GT1_OUT_W_kgps/1, G02_GT1_OUT_W_kgps/1, Scope_G01_G08/2
  P4/1 -> 截面输入展开/8(P4_Pa)
  全局保护参数/1(GlobalParams7) -> G08_动力涡轮二级叶尖出口/3(GlobalParams7), G05_动力涡轮一级叶根进口/3(GlobalParams7), G06_动力涡轮一级叶根出口/3(GlobalParams7), G02_燃气涡轮一级出口/3(GlobalParams7), G01_燃气涡轮一级进口/3(GlobalParams7), G03_燃气涡轮二级进口/3(GlobalParams7), G07_动力涡轮二级叶尖进口/3(GlobalParams7), G04_燃气涡轮二级出口/3(GlobalParams7)
  T45/1 -> 截面输入展开/9(T45_K)
  T5/1 -> 截面输入展开/11(T5_K)
  P25/1 -> 截面输入展开/6(P3_Pa)
  G08_动力涡轮二级叶尖出口/1(G08_PT2_OUT_TIP_W_kgps) -> Scope_G01_G08/8, Scope_G08_PT2_OUT_TIP_W_kgps/1, G08_PT2_OUT_TIP_W_kgps/1
  G05_动力涡轮一级叶根进口/1(G05_PT1_IN_ROOT_W_kgps) -> Scope_G01_G08/5, G05_PT1_IN_ROOT_W_kgps/1, Scope_G05_PT1_IN_ROOT_W_kgps/1
  G06_动力涡轮一级叶根出口/1(G06_PT1_OUT_ROOT_W_kgps) -> Scope_G01_G08/6, Scope_G06_PT1_OUT_ROOT_W_kgps/1, G06_PT1_OUT_ROOT_W_kgps/1
  截面输入展开/1(BoundaryTP24) -> G07_动力涡轮二级叶尖进口/1(BoundaryTP24), G06_动力涡轮一级叶根出口/1(BoundaryTP24), G08_动力涡轮二级叶尖出口/1(BoundaryTP24), G05_动力涡轮一级叶根进口/1(BoundaryTP24), G02_燃气涡轮一级出口/1(BoundaryTP24), G03_燃气涡轮二级进口/1(BoundaryTP24), G01_燃气涡轮一级进口/1(BoundaryTP24), G04_燃气涡轮二级出口/1(BoundaryTP24)
  G04_燃气涡轮二级出口/1(G04_GT2_OUT_W_kgps) -> Scope_G01_G08/4, G04_GT2_OUT_W_kgps/1, Scope_G04_GT2_OUT_W_kgps/1
  G01_燃气涡轮一级进口/1(G01_GT1_IN_W_kgps) -> Scope_G01_G08/1, Scope_G01_GT1_IN_W_kgps/1, G01_GT1_IN_W_kgps/1
  NG/1 -> G02_燃气涡轮一级出口/2(RotorSpeed_rpm), G04_燃气涡轮二级出口/2(RotorSpeed_rpm), G03_燃气涡轮二级进口/2(RotorSpeed_rpm), G01_燃气涡轮一级进口/2(RotorSpeed_rpm)
  G03_燃气涡轮二级进口/1(G03_GT2_IN_W_kgps) -> Scope_G01_G08/3, Scope_G03_GT2_IN_W_kgps/1, G03_GT2_IN_W_kgps/1
  NP/1 -> G05_动力涡轮一级叶根进口/2(RotorSpeed_rpm), G07_动力涡轮二级叶尖进口/2(RotorSpeed_rpm), G06_动力涡轮一级叶根出口/2(RotorSpeed_rpm), G08_动力涡轮二级叶尖出口/2(RotorSpeed_rpm)
  G07_动力涡轮二级叶尖进口/1(G07_PT2_IN_TIP_W_kgps) -> Scope_G01_G08/7, G07_PT2_IN_TIP_W_kgps/1, Scope_G07_PT2_IN_TIP_W_kgps/1
  T4/1 -> 截面输入展开/7(T4_K)
  P5/1 -> 截面输入展开/12(P45_Pa)
  T25/1 -> 截面输入展开/5(T3_K)
  25/1 -> Demux_SFuncAirPerfRows/1
  Demux_SFuncAirPerfRows/1 -> 截面输入展开/3(T252_K)
  Demux_SFuncAirPerfRows/4 -> 截面输入展开/2(P251_Pa)
  Demux_SFuncAirPerfRows/2 -> 截面输入展开/4(P252_Pa)
  Demux_SFuncAirPerfRows/3 -> 截面输入展开/1(T251_K)
  G04_燃气涡轮二级出口/2(G04_Supply_T_K) -> G04_Supply_T_K/1
  G04_燃气涡轮二级出口/3(G04_Supply_P_Pa) -> G04_Supply_P_Pa/1

== system Dll_Control_AFO_V8_5_R2019b/滑油系统代理模型/AB轴承腔通风模块 ==
  VentBoundary10 : Inport  PortDimensions=10
  RotorSpeed2 : Inport  Port=2  PortDimensions=2
  四封严双腔通风计算 : MATLAB Function  TreatAsAtomicUnit=on
  CavityState8_PaK : Outport  PortDimensions=8
  SealLeak4_kgps : Outport  Port=2  PortDimensions=4
  VentFlow3_kgps : Outport  Port=3  PortDimensions=3
  SealDeltaP4_Pa : Outport  Port=4  PortDimensions=4
  VentDeltaP2_Pa : Outport  Port=5  PortDimensions=2
  MassResidual2_kgps : Outport  Port=6  PortDimensions=2
  wires:
  四封严双腔通风计算/4(sealDP4) -> SealDeltaP4_Pa/1
  四封严双腔通风计算/5(ventDP2) -> VentDeltaP2_Pa/1
  四封严双腔通风计算/6(residual2) -> MassResidual2_kgps/1
  VentBoundary10/1 -> 四封严双腔通风计算/1(boundary10)
  RotorSpeed2/1 -> 四封严双腔通风计算/2(speed2)
  四封严双腔通风计算/1(cavityState8) -> CavityState8_PaK/1
  四封严双腔通风计算/2(leak4) -> SealLeak4_kgps/1
  四封严双腔通风计算/3(vent3) -> VentFlow3_kgps/1

== system Dll_Control_AFO_V8_5_R2019b/滑油系统代理模型/AMESim_滑油泵转速流量 ==
  note: Qpump = 0.46751 × 2.5 × 0.358 × Ng / 1000；设计点 38000 rpm → 15.9 L/min
  Ng_rpm : Inport
  泵排量_cc_rev : Inport  Port=2
  cc_rev_to_L_min : Gain  Gain=1/1000
  传动比_AMESim : Gain  Gain=0.358
  排量有效选择 : Switch  Threshold=0.1
  有效容积系数 : Gain  Gain=0.467509556012937
  流量保护 : Saturate  UpperLimit=45  LowerLimit=0
  转速乘排量 : Product  Inputs=**
  默认排量 : Constant  Value=2.5
  Qpump_L_min : Outport
  wires:
  Ng_rpm/1 -> 传动比_AMESim/1
  传动比_AMESim/1 -> 转速乘排量/1
  泵排量_cc_rev/1 -> 排量有效选择/1, 排量有效选择/2
  默认排量/1 -> 排量有效选择/3
  排量有效选择/1 -> 转速乘排量/2
  转速乘排量/1 -> cc_rev_to_L_min/1
  cc_rev_to_L_min/1 -> 有效容积系数/1
  有效容积系数/1 -> 流量保护/1
  流量保护/1 -> Qpump_L_min/1  "Qpump_L_min"

== system Dll_Control_AFO_V8_5_R2019b/滑油系统代理模型/散热器模块 ==
  OilInlet2_C : Inport  PortDimensions=2
  燃滑空滑特性 : MATLAB Function  TreatAsAtomicUnit=on
  FuelOil2_ToutC_QkW : Outport  PortDimensions=2
  AirOil2_ToutC_QkW : Outport  Port=2  PortDimensions=2
  wires:
  OilInlet2_C/1 -> 燃滑空滑特性/1(oilInlet2C)
  燃滑空滑特性/1(fuel2) -> FuelOil2_ToutC_QkW/1
  燃滑空滑特性/2(air2) -> AirOil2_ToutC_QkW/1

== system Dll_Control_AFO_V8_5_R2019b/滑油系统代理模型/滑油系统代理核心 ==
  输入向量 : Inport  PortDimensions=26
  支路_流量压力分配 : Subsystem
  支路_燃滑散热 : Subsystem
  支路_空滑换热 : Subsystem
  支路_轴承甲乙换热 : Subsystem
  支路机匣附件换热 : Subsystem
  甲轴承腔换热量 : Outport
  乙轴承腔换热量 : Outport  Port=2
  空滑换热量 : Outport  Port=3
  机匣附件换热量 : Outport  Port=4
  甲轴承腔流量 : Outport  Port=5
  乙轴承腔流量 : Outport  Port=6
  甲轴承腔压力 : Outport  Port=7
  乙轴承腔压力 : Outport  Port=8
  甲轴承腔出口油温 : Outport  Port=9
  乙轴承腔出口油温 : Outport  Port=10
  A腔回油流量 : Outport  Port=11
  B腔回油流量 : Outport  Port=12
  甲轴承腔生热量 : Outport  Port=13
  乙轴承腔生热量 : Outport  Port=14
  FuelOilCooler_Q : Outport  Port=15
  FuelOilCooler_FuelTout : Outport  Port=16
  AirOilCooler_Pin_Pa : Outport  Port=17
  AirOilCooler_Pout_Pa : Outport  Port=18
  FuelOilCooler_Pin_Pa : Outport  Port=19
  FuelOilCooler_Pout_Pa : Outport  Port=20
  wires:
  支路_流量压力分配/6(B腔回油流量) -> B腔回油流量/1, 支路_空滑换热/3(QretB_m3_s)
  支路_轴承甲乙换热/3(甲轴承腔出口油温) -> 甲轴承腔出口油温/1
  支路_燃滑散热/1(FuelOilCooler_Q) -> FuelOilCooler_Q/1
  支路_轴承甲乙换热/1(甲轴承腔换热量) -> 甲轴承腔换热量/1
  支路_流量压力分配/7(QG_m3_s) -> 支路_燃滑散热/4(QG_m3_s)
  支路_流量压力分配/9(Pret_Pa) -> 支路_空滑换热/4(Pret_Pa)
  输入向量/1 -> 支路_轴承甲乙换热/1(输入向量), 支路_空滑换热/1(输入向量), 支路_流量压力分配/1(输入向量), 支路机匣附件换热/1(输入向量), 支路_燃滑散热/1(输入向量)
  支路_流量压力分配/8(Pman_Pa) -> 支路_燃滑散热/5(Pman_Pa)
  支路_流量压力分配/4(乙轴承腔压力) -> 乙轴承腔压力/1, 支路_燃滑散热/7(PB_Pa)
  支路_空滑换热/2(AirOilCooler_Pin_Pa) -> AirOilCooler_Pin_Pa/1
  支路_燃滑散热/2(FuelOilCooler_FuelTout) -> FuelOilCooler_FuelTout/1
  支路_轴承甲乙换热/2(乙轴承腔换热量) -> 乙轴承腔换热量/1
  支路_燃滑散热/3(FuelOilCooler_Pin_Pa) -> FuelOilCooler_Pin_Pa/1
  支路_轴承甲乙换热/6(乙轴承腔生热量) -> 乙轴承腔生热量/1
  支路_轴承甲乙换热/4(乙轴承腔出口油温) -> 乙轴承腔出口油温/1
  支路_空滑换热/1(空滑换热量) -> 空滑换热量/1
  支路_燃滑散热/4(FuelOilCooler_Pout_Pa) -> FuelOilCooler_Pout_Pa/1
  支路机匣附件换热/1(机匣附件换热量) -> 机匣附件换热量/1
  支路_流量压力分配/3(甲轴承腔压力) -> 甲轴承腔压力/1, 支路_燃滑散热/6(PA_Pa)
  支路_空滑换热/3(AirOilCooler_Pout_Pa) -> AirOilCooler_Pout_Pa/1
  支路_轴承甲乙换热/5(甲轴承腔生热量) -> 甲轴承腔生热量/1
  支路_流量压力分配/1(甲轴承腔流量) -> 甲轴承腔流量/1, 支路_燃滑散热/2(QA_m3_s)
  支路_流量压力分配/2(乙轴承腔流量) -> 乙轴承腔流量/1, 支路_燃滑散热/3(QB_m3_s)
  支路_流量压力分配/5(A腔回油流量) -> A腔回油流量/1, 支路_空滑换热/2(QretA_m3_s)

== system Dll_Control_AFO_V8_5_R2019b/燃油系统代理模型1/Signal Builder ==
  Demux : Demux  Tag=STV Demux  Outputs=1
  FromWs : FromWorkspace  Tag=STV FromWs  VariableName=tuvar  SampleTime=0
      SigBuilderData=|
      | common.afterFinalStr = 'Extrapolate'
      | common.sampleTime = 0
      | dataSet.timeRange = [0 10]
      | dataSet.name = 'Group 1'
      | sbobj.Groups.Name = 'Group 1'
      | sbobj.Groups.Signals.Name = 'Signal 1'
      | sbobj.Groups.Signals.XData = [0 1 1 2 2 3 3 4 4 5 5 6 6 7 7 10]
      | sbobj.Groups.Signals.YData = [0 0 0.00075 0.00075 0.00185 0.00185 0.008 0.008 0.0098 0.0098 0.008 0.008 0.006 0.006 0 0]
  Signal 1 : Outport  Tag=STV Outport
  wires:
  Demux/1 -> Signal 1/1
  FromWs/1 -> Demux/1

== system Dll_Control_AFO_V8_5_R2019b/燃油系统代理模型1/Signal Builder1 ==
  Demux : Demux  Tag=STV Demux  Outputs=1
  FromWs : FromWorkspace  Tag=STV FromWs  VariableName=tuvar  SampleTime=0
      SigBuilderData=|
      | common.afterFinalStr = 'Extrapolate'
      | common.sampleTime = 0
      | dataSet.timeRange = [0 10]
      | dataSet.name = 'Group 1'
      | sbobj.Groups.Name = 'Group 1'
      | sbobj.Groups.Signals.Name = 'Signal 1'
      | sbobj.Groups.Signals.XData = [0 2 2 4 4 6 6 8 8 10]
      | sbobj.Groups.Signals.YData = [0 0 0.015 0.015 0.03 0.03 0.05 0.05 0 0]
  Signal 1 : Outport  Tag=STV Outport
  wires:
  Demux/1 -> Signal 1/1
  FromWs/1 -> Demux/1

== system Dll_Control_AFO_V8_5_R2019b/燃油系统代理模型1/Wf_to_xm_inverse ==
  Wf_cmd_kgps : Inport
  Kgps2Lmin_Gain : Gain  Gain=60000/780
  Wf2xm_Gain : Gain  Gain=(1e-3/60)/(0.7*0.00094*sqrt(2*0.38*1e6/780))
  xm_Sat : Saturate  UpperLimit=0.012  LowerLimit=0
  xm_cmd_m : Outport
  wires:
  Wf_cmd_kgps/1 -> Kgps2Lmin_Gain/1
  Kgps2Lmin_Gain/1 -> Wf2xm_Gain/1
  Wf2xm_Gain/1 -> xm_Sat/1
  xm_Sat/1 -> xm_cmd_m/1

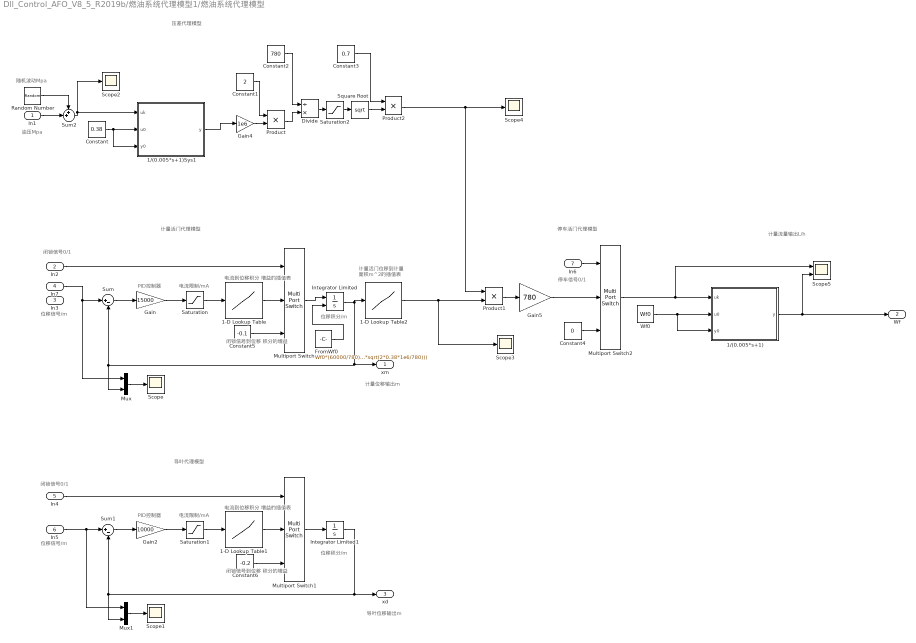
== system Dll_Control_AFO_V8_5_R2019b/燃油系统代理模型1/燃油系统代理模型 ==
  note: 计量活门代理模型
  note: PID控制器
  note: 电流限制/mA
  note: 电流到位移积分
      | 增益的插值表
  note: 位移积分/m
  note: 位移信号/m
  note: 闭锁信号0/1
  note: 闭锁信号到位移
      | 积分的增益
  note: 导叶代理模型
  note: 位移信号/m
  note: 闭锁信号0/1
  note: 电流到位移积分
      | 增益的插值表
  note: 位移积分/m
  note: 电流限制/mA
  note: 闭锁信号到位移
      | 积分的增益
  note: PID控制器
  note: 计量活门位移到计量
      | 面积m^2的插值表
  note: 油压Mpa
  note: 压差代理模型
  note: 随机波动Mpa
  note: 停车信号0/1
  note: 停车活门代理模型
  note: 计量流量输出L/h
  note: 计量位移输出m
  note: 导叶位移输出m
  In1 : Inport
  In2 : Inport  Port=2
  In3 : Inport  Port=3
  In7 : Inport  Port=4
  In4 : Inport  Port=5
  In5 : Inport  Port=6
  In6 : Inport  Port=7
  1-D Lookup Table : Lookup_n-D  NumberOfTableDimensions=1  BreakpointsForDimension1=[-40 0 40]  Table=[-0.08 0 0.08]  InternalRulePriority=Speed  RndMeth=Simplest  InputSameDT=on
  1-D Lookup Table1 : Lookup_n-D  NumberOfTableDimensions=1  BreakpointsForDimension1=[-40 0 40]  Table=[-0.12 0 0.12]  InternalRulePriority=Speed  RndMeth=Simplest  InputSameDT=on
  1-D Lookup Table2 : Lookup_n-D  NumberOfTableDimensions=1  BreakpointsForDimension1=[0 0.006 0.012]  Table=[0 0.006 0.012]*0.00094  InternalRulePriority=Speed  RndMeth=Simplest  InputSameDT=on
  1/(0.005*s+1) : Subsystem
  1/(0.005*s+1)Sys1 : Subsystem
  Constant : Constant  Value=0.38
  Constant1 : Constant  Value=2
  Constant2 : Constant  Value=780
  Constant3 : Constant  Value=0.7
  Constant4 : Constant  Value=0
  Constant5 : Constant  Value=-0.1
  Constant6 : Constant  Value=-0.2
  Divide : Product  Inputs=/*
  FromWf0 : Constant  Value=Wf0*(60000/780)*((1e-3/60)/(0.7*0.00094*sqrt(2*0.38*1e6/780)))
  Gain : Gain  Gain=15000
  Gain2 : Gain  Gain=10000
  Gain4 : Gain  Gain=1e6
  Gain5 : Gain  Gain=780
  Integrator Limited : Integrator  InitialConditionSource=external  LimitOutput=on  UpperSaturationLimit=0.012  LowerSaturationLimit=0
  Integrator Limited1 : Integrator  LimitOutput=on  UpperSaturationLimit=0.05  LowerSaturationLimit=0
  Multiport Switch : MultiPortSwitch  DataPortOrder=Zero-based contiguous  Inputs=2  zeroidx=on
  Multiport Switch1 : MultiPortSwitch  DataPortOrder=Zero-based contiguous  Inputs=2  zeroidx=on
  Multiport Switch2 : MultiPortSwitch  DataPortOrder=Zero-based contiguous  Inputs=2  zeroidx=on
  Mux : Mux  Inputs=2
  Mux1 : Mux  Inputs=2
  Product : Product
  Product1 : Product
  Product2 : Product
  Random Number : RandomNumber  Variance=1e-5*0  SampleTime=Ts
  Saturation : Saturate  UpperLimit=40  LowerLimit=-40
  Saturation1 : Saturate  UpperLimit=40  LowerLimit=-40
  Saturation2 : Saturate  UpperLimit=1e10  LowerLimit=0
  Scope{,1..4} (5 alike) : Scope
  Scope5 : Scope  NumInputPorts=2
  Square Root : Sqrt  SaturateOnIntegerOverflow=on
  Sum : Sum  Inputs=|+-
  Sum1 : Sum  Inputs=|+-
  Sum2 : Sum  Inputs=++|
  Wf0 : Constant  Value=Wf0
  xm : Outport
  Wf : Outport  Port=2
  xd : Outport  Port=3
  wires:
  Integrator Limited1/1 -> xd/1, Sum1/2, Mux1/2
  Constant5/1 -> Multiport Switch/3
  Integrator Limited/1 -> 1-D Lookup Table2/1, xm/1, Sum/2, Mux/2
  1-D Lookup Table1/1 -> Multiport Switch1/2
  1-D Lookup Table/1 -> Multiport Switch/2
  Multiport Switch1/1 -> Integrator Limited1/1
  Divide/1 -> Saturation2/1
  Gain2/1 -> Saturation1/1
  Constant1/1 -> Product/1
  In4/1 -> Multiport Switch1/1
  Mux1/1 -> Scope1/1
  In5/1 -> Mux1/1, Sum1/1
  Saturation1/1 -> 1-D Lookup Table1/1
  Sum1/1 -> Gain2/1
  Constant6/1 -> Multiport Switch1/3
  Mux/1 -> Scope/1
  Product/1 -> Divide/2
  Product2/1 -> Product1/1, Scope4/1
  Constant3/1 -> Product2/1
  In6/1 -> Multiport Switch2/1
  Sum/1 -> Gain/1
  Gain/1 -> Saturation/1
  Saturation/1 -> 1-D Lookup Table/1
  Constant4/1 -> Multiport Switch2/3
  Constant2/1 -> Divide/1
  In2/1 -> Multiport Switch/1
  1-D Lookup Table2/1 -> Scope3/1, Product1/2
  Multiport Switch/1 -> Integrator Limited/1
  Product1/1 -> Gain5/1
  Square Root/1 -> Product2/2
  In1/1 -> Sum2/2
  Saturation2/1 -> Square Root/1
  Gain4/1 -> Product/2
  Sum2/1 -> Scope2/1, 1/(0.005*s+1)Sys1/1(uk)
  FromWf0/1 -> Integrator Limited/2
  Gain5/1 -> Multiport Switch2/2
  Random Number/1 -> Sum2/1
  Multiport Switch2/1 -> Scope5/1, 1/(0.005*s+1)/1(uk)
  1/(0.005*s+1)/1(y) -> Scope5/2, Wf/1
  Wf0/1 -> 1/(0.005*s+1)/3(y0), 1/(0.005*s+1)/2(u0)
  Constant/1 -> 1/(0.005*s+1)Sys1/3(y0), 1/(0.005*s+1)Sys1/2(u0)
  1/(0.005*s+1)Sys1/1(y) -> Gain4/1
  In7/1 -> Mux/1, Sum/1

== system Dll_Control_AFO_V8_5_R2019b/空气系统代理模型/G01_燃气涡轮一级进口 ==
  BoundaryTP24 : Inport  PortDimensions=24
  RotorSpeed_rpm : Inport  Port=2  PortDimensions=1
  GlobalParams7 : Inport  Port=3  PortDimensions=7
  EffectiveAreaScale : Selector  InputPortWidth=7  IndexOptions=Index vector (dialog)  Indices=1  OutputSizes=1
  SealCorrection : Selector  InputPortWidth=7  IndexOptions=Index vector (dialog)  Indices=7  OutputSizes=1
  可压缩节流孔口 : Subsystem  Description=Embedded ideal-gas compressible restrictor with critical pressure ratio. No external MATLAB runtime function.  mask{UpstreamBoundary=10, DownstreamBoundary=1}
      mask prompts: UpstreamBoundary "Upstream boundary index"; DownstreamBoundary "Downstream boundary index"
  导叶冷却 : Gain  Gain=0.90000000000000002
  未用转速终止 : Terminator
  流路可调参数 : Subsystem  Description=流路级可调物理参数（已内置在 SLX）。
  流量物理限幅 : Saturate  UpperLimit=2  LowerLimit=0
  盘腔热动态 : Subsystem  Description=Embedded discrete first-order lag with exact bypass when tau is zero.  mask{SampleTime_s=0.025000000000000001, InitialFlowValue=0.54362352012440196}
      mask prompts: SampleTime_s "Sample time [s]"; InitialFlowValue "Initial output [kg/s]"
  等效面积缩放 : Product  Inputs=**
  篦齿修正 : Product  Inputs=**
  辨识等效面积 : Subsystem  Description=辨识得到的等效面积律（内嵌 MATLAB Function）。
  G01_GT1_IN_W_kgps : Outport
  wires:
  流量物理限幅/1 -> G01_GT1_IN_W_kgps/1
  可压缩节流孔口/1(W_kgps) -> 导叶冷却/1
  盘腔热动态/1(W_out) -> 流量物理限幅/1
  篦齿修正/1 -> 盘腔热动态/1(W_in)
  SealCorrection/1 -> 篦齿修正/2
  导叶冷却/1 -> 篦齿修正/1
  RotorSpeed_rpm/1 -> 未用转速终止/1
  GlobalParams7/1 -> 可压缩节流孔口/3(GlobalParams7)
  等效面积缩放/1 -> 可压缩节流孔口/2(EffectiveArea_m2)
  BoundaryTP24/1 -> 辨识等效面积/1(BoundaryTP24), 可压缩节流孔口/1(BoundaryTP24)
  EffectiveAreaScale/1 -> 等效面积缩放/2
  辨识等效面积/1(EffectiveArea_m2) -> 等效面积缩放/1
  流路可调参数/1(RouteParams7) -> EffectiveAreaScale/1, 盘腔热动态/2(RouteParams7), SealCorrection/1

== system Dll_Control_AFO_V8_5_R2019b/空气系统代理模型/G02_燃气涡轮一级出口 ==
  BoundaryTP24 : Inport  PortDimensions=24
  RotorSpeed_rpm : Inport  Port=2  PortDimensions=1
  GlobalParams7 : Inport  Port=3  PortDimensions=7
  EffectiveAreaScale : Selector  InputPortWidth=7  IndexOptions=Index vector (dialog)  Indices=1  OutputSizes=1
  SealCorrection : Selector  InputPortWidth=7  IndexOptions=Index vector (dialog)  Indices=7  OutputSizes=1
  可压缩节流孔口 : Subsystem  Description=Embedded ideal-gas compressible restrictor with critical pressure ratio. No external MATLAB runtime function.  mask{UpstreamBoundary=12, DownstreamBoundary=2}
      mask prompts: UpstreamBoundary "Upstream boundary index"; DownstreamBoundary "Downstream boundary index"
  旋转离心压升 : Subsystem  Description=Embedded centrifugal pressure rise: 0.5*kRot*rho*omega^2*(rOut^2-rIn^2).  mask{UpstreamBoundary=12, DownstreamBoundary=2}
      mask prompts: UpstreamBoundary "Upstream boundary index"; DownstreamBoundary "Downstream boundary index"
  机匣冷却 : Gain  Gain=0.92000000000000004
  流路可调参数 : Subsystem  Description=流路级可调物理参数（已内置在 SLX）。
  流量物理限幅 : Saturate  UpperLimit=2  LowerLimit=0
  盘腔热动态 : Subsystem  Description=Embedded discrete first-order lag with exact bypass when tau is zero.  mask{SampleTime_s=0.025000000000000001, InitialFlowValue=0.20536888538032999}
      mask prompts: SampleTime_s "Sample time [s]"; InitialFlowValue "Initial output [kg/s]"
  等效面积缩放 : Product  Inputs=**
  篦齿修正 : Product  Inputs=**
  篦齿封严 : Gain  Gain=0.88
  辨识等效面积 : Subsystem  Description=辨识得到的等效面积律（内嵌 MATLAB Function）。
  G02_GT1_OUT_W_kgps : Outport
  wires:
  流量物理限幅/1 -> G02_GT1_OUT_W_kgps/1
  盘腔热动态/1(W_out) -> 流量物理限幅/1
  篦齿封严/1 -> 篦齿修正/1
  等效面积缩放/1 -> 可压缩节流孔口/2(EffectiveArea_m2)
  篦齿修正/1 -> 盘腔热动态/1(W_in)
  SealCorrection/1 -> 篦齿修正/2
  机匣冷却/1 -> 篦齿封严/1
  旋转离心压升/1(W_out) -> 机匣冷却/1
  RotorSpeed_rpm/1 -> 旋转离心压升/3(RotorSpeed_rpm)
  BoundaryTP24/1 -> 可压缩节流孔口/1(BoundaryTP24), 旋转离心压升/2(BoundaryTP24), 辨识等效面积/1(BoundaryTP24)
  可压缩节流孔口/1(W_kgps) -> 旋转离心压升/1(W_in)
  GlobalParams7/1 -> 可压缩节流孔口/3(GlobalParams7), 旋转离心压升/4(GlobalParams7)
  EffectiveAreaScale/1 -> 等效面积缩放/2
  辨识等效面积/1(EffectiveArea_m2) -> 等效面积缩放/1
  流路可调参数/1(RouteParams7) -> SealCorrection/1, 盘腔热动态/2(RouteParams7), 旋转离心压升/5(RouteParams7), EffectiveAreaScale/1

== system Dll_Control_AFO_V8_5_R2019b/空气系统代理模型/G03_燃气涡轮二级进口 ==
  BoundaryTP24 : Inport  PortDimensions=24
  RotorSpeed_rpm : Inport  Port=2  PortDimensions=1
  GlobalParams7 : Inport  Port=3  PortDimensions=7
  EffectiveAreaScale : Selector  InputPortWidth=7  IndexOptions=Index vector (dialog)  Indices=1  OutputSizes=1
  SealCorrection : Selector  InputPortWidth=7  IndexOptions=Index vector (dialog)  Indices=7  OutputSizes=1
  可压缩节流孔口 : Subsystem  Description=Embedded ideal-gas compressible restrictor with critical pressure ratio. No external MATLAB runtime function.  mask{UpstreamBoundary=10, DownstreamBoundary=3}
      mask prompts: UpstreamBoundary "Upstream boundary index"; DownstreamBoundary "Downstream boundary index"
  导叶冷却 : Gain  Gain=0.90000000000000002
  旋转离心压升 : Subsystem  Description=Embedded centrifugal pressure rise: 0.5*kRot*rho*omega^2*(rOut^2-rIn^2).  mask{UpstreamBoundary=10, DownstreamBoundary=3}
      mask prompts: UpstreamBoundary "Upstream boundary index"; DownstreamBoundary "Downstream boundary index"
  流路可调参数 : Subsystem  Description=流路级可调物理参数（已内置在 SLX）。
  流量物理限幅 : Saturate  UpperLimit=2  LowerLimit=0
  盘腔热动态 : Subsystem  Description=Embedded discrete first-order lag with exact bypass when tau is zero.  mask{SampleTime_s=0.025000000000000001, InitialFlowValue=0.165771616630528}
      mask prompts: SampleTime_s "Sample time [s]"; InitialFlowValue "Initial output [kg/s]"
  等效面积缩放 : Product  Inputs=**
  篦齿修正 : Product  Inputs=**
  辨识等效面积 : Subsystem  Description=辨识得到的等效面积律（内嵌 MATLAB Function）。
  G03_GT2_IN_W_kgps : Outport
  wires:
  EffectiveAreaScale/1 -> 等效面积缩放/2
  流量物理限幅/1 -> G03_GT2_IN_W_kgps/1
  盘腔热动态/1(W_out) -> 流量物理限幅/1
  篦齿修正/1 -> 盘腔热动态/1(W_in)
  等效面积缩放/1 -> 可压缩节流孔口/2(EffectiveArea_m2)
  SealCorrection/1 -> 篦齿修正/2
  导叶冷却/1 -> 篦齿修正/1
  旋转离心压升/1(W_out) -> 导叶冷却/1
  RotorSpeed_rpm/1 -> 旋转离心压升/3(RotorSpeed_rpm)
  可压缩节流孔口/1(W_kgps) -> 旋转离心压升/1(W_in)
  辨识等效面积/1(EffectiveArea_m2) -> 等效面积缩放/1
  GlobalParams7/1 -> 可压缩节流孔口/3(GlobalParams7), 旋转离心压升/4(GlobalParams7)
  BoundaryTP24/1 -> 可压缩节流孔口/1(BoundaryTP24), 旋转离心压升/2(BoundaryTP24), 辨识等效面积/1(BoundaryTP24)
  流路可调参数/1(RouteParams7) -> SealCorrection/1, 盘腔热动态/2(RouteParams7), 旋转离心压升/5(RouteParams7), EffectiveAreaScale/1

== system Dll_Control_AFO_V8_5_R2019b/空气系统代理模型/G04_燃气涡轮二级出口 ==
  BoundaryTP24 : Inport  PortDimensions=24
  RotorSpeed_rpm : Inport  Port=2  PortDimensions=1
  GlobalParams7 : Inport  Port=3  PortDimensions=7
  EffectiveAreaScale : Selector  InputPortWidth=7  IndexOptions=Index vector (dialog)  Indices=1  OutputSizes=1
  SealCorrection : Selector  InputPortWidth=7  IndexOptions=Index vector (dialog)  Indices=7  OutputSizes=1
  Selector_G04_Supply_P_Pa : Selector  InputPortWidth=24  IndexOptions=Index vector (dialog)  Indices=24  OutputSizes=1
  Selector_G04_Supply_T_K : Selector  InputPortWidth=24  IndexOptions=Index vector (dialog)  Indices=23  OutputSizes=1
  可压缩节流孔口 : Subsystem  Description=Embedded ideal-gas compressible restrictor with critical pressure ratio. No external MATLAB runtime function.  mask{UpstreamBoundary=12, DownstreamBoundary=4}
      mask prompts: UpstreamBoundary "Upstream boundary index"; DownstreamBoundary "Downstream boundary index"
  旋转离心压升 : Subsystem  Description=Embedded centrifugal pressure rise: 0.5*kRot*rho*omega^2*(rOut^2-rIn^2).  mask{UpstreamBoundary=12, DownstreamBoundary=4}
      mask prompts: UpstreamBoundary "Upstream boundary index"; DownstreamBoundary "Downstream boundary index"
  机匣冷却 : Gain  Gain=0.92000000000000004
  流路可调参数 : Subsystem  Description=流路级可调物理参数（已内置在 SLX）。
  流量物理限幅 : Saturate  UpperLimit=2  LowerLimit=0
  等效面积缩放 : Product  Inputs=**
  篦齿修正 : Product  Inputs=**
  篦齿封严 : Gain  Gain=0.88
  辨识等效面积 : Subsystem  Description=辨识得到的等效面积律（内嵌 MATLAB Function）。
  G04_GT2_OUT_W_kgps : Outport
  G04_Supply_T_K : Outport  Port=2
  G04_Supply_P_Pa : Outport  Port=3
  wires:
  EffectiveAreaScale/1 -> 等效面积缩放/2
  流量物理限幅/1 -> G04_GT2_OUT_W_kgps/1
  篦齿修正/1 -> 流量物理限幅/1
  篦齿封严/1 -> 篦齿修正/1
  SealCorrection/1 -> 篦齿修正/2
  机匣冷却/1 -> 篦齿封严/1
  GlobalParams7/1 -> 可压缩节流孔口/3(GlobalParams7), 旋转离心压升/4(GlobalParams7)
  旋转离心压升/1(W_out) -> 机匣冷却/1
  辨识等效面积/1(EffectiveArea_m2) -> 等效面积缩放/1
  等效面积缩放/1 -> 可压缩节流孔口/2(EffectiveArea_m2)
  RotorSpeed_rpm/1 -> 旋转离心压升/3(RotorSpeed_rpm)
  可压缩节流孔口/1(W_kgps) -> 旋转离心压升/1(W_in)
  BoundaryTP24/1 -> 可压缩节流孔口/1(BoundaryTP24), 旋转离心压升/2(BoundaryTP24), 辨识等效面积/1(BoundaryTP24), Selector_G04_Supply_T_K/1, Selector_G04_Supply_P_Pa/1
  流路可调参数/1(RouteParams7) -> SealCorrection/1, 旋转离心压升/5(RouteParams7), EffectiveAreaScale/1
  Selector_G04_Supply_T_K/1 -> G04_Supply_T_K/1
  Selector_G04_Supply_P_Pa/1 -> G04_Supply_P_Pa/1
